simulink subsystem "Integrator_dyn_sat"  (R2022b)
settings: Solver=VariableStepAuto  StartTime=0.0  StopTime=10.0  RelTol=1e-3
model mask{initValue=0, T_s=-1}
undefined symbols (not defined in the file or in its folder): DiscIntNeverNeededParam
libraries: simulink x10
settings Model: Creator=winkens  LastModifiedBy=winkens
settings SolverCC: AlgebraicLoopSolver=TrustRegion
settings DebuggingCC: UnconnectedInputMsg=warning  UnconnectedOutputMsg=warning  UnconnectedLineMsg=warning  SFMachineParentedDataDiag=warning
settings ModelReferenceCC: EnableRefExpFcnMdlSchedulingChecks=on
settings RTWCC: DLArmComputeVersion=19.05

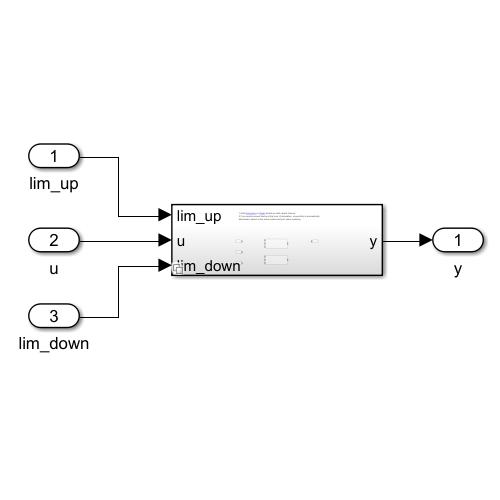
[thumbnail: Simulink's stored preview of the top-level diagram]
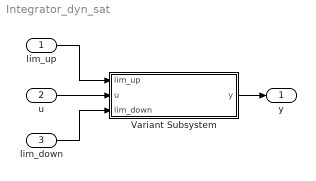
== system Integrator_dyn_sat ==
  lim_up : Inport
  u : Inport  Port=2
  lim_down : Inport  Port=3
  Variant Subsystem : Subsystem  Variant=on
  y : Outport
  wires:
  lim_up/1 -> Variant Subsystem/1(lim_up)
  lim_down/1 -> Variant Subsystem/3(lim_down)
  u/1 -> Variant Subsystem/2(u)
  Variant Subsystem/1(y) -> y/1

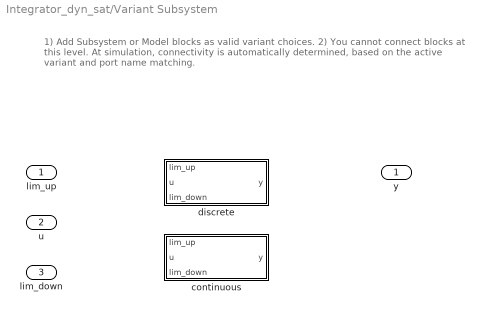
== system Integrator_dyn_sat/Variant Subsystem ==
  note: 1) Add Subsystem or Model blocks as valid variant choices.
      | 2) You cannot connect blocks at this level. At simulation, connectivity is automatically
      | determined, based on the active variant and port name matching.
  lim_up : Inport
  u : Inport  Port=2
  lim_down : Inport  Port=3
  continuous : Subsystem  VariantControl=T_s == 0
  discrete : Subsystem  VariantControl=(default)
  y : Outport

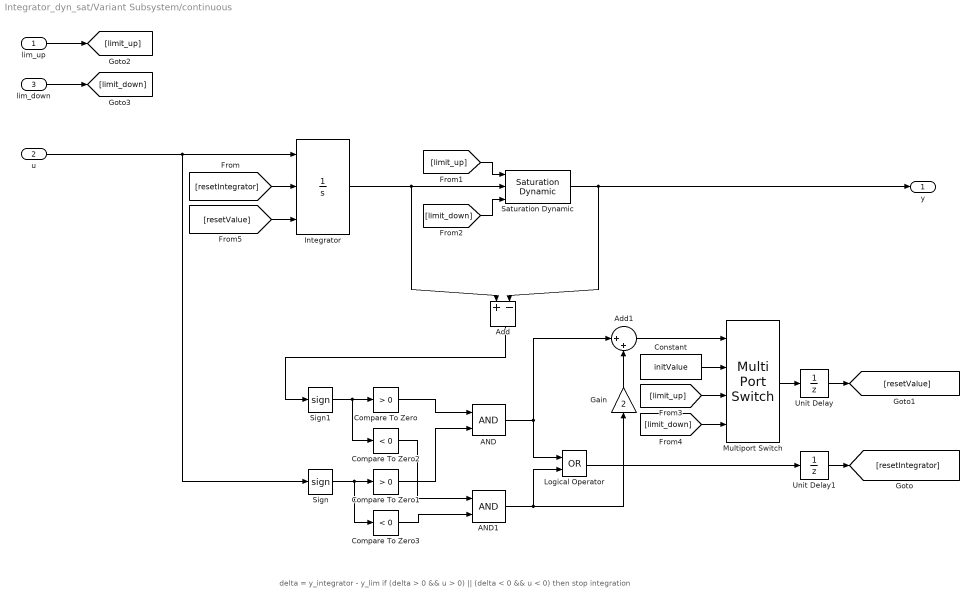
== system Integrator_dyn_sat/Variant Subsystem/continuous ==
  note: delta = y_integrator - y_lim
      |
      | if (delta > 0 && u > 0) || (delta < 0 && u < 0) then stop integration
  lim_up : Inport
  u : Inport  Port=2
  lim_down : Inport  Port=3
  AND : Logic  AllPortsSameDT=off  OutDataTypeStr=boolean
  AND1 : Logic  AllPortsSameDT=off  OutDataTypeStr=boolean
  Add : Sum  Inputs=+-
  Add1 : Sum  Inputs=|++
  Compare To Zero : simulink/Logic and Bit Operations/Compare To Zero  relop=>  OutDataTypeStr=boolean
  Compare To Zero1 : simulink/Logic and Bit Operations/Compare To Zero  relop=>  OutDataTypeStr=boolean
  Compare To Zero2 : simulink/Logic and Bit Operations/Compare To Zero  relop=<  OutDataTypeStr=boolean
  Compare To Zero3 : simulink/Logic and Bit Operations/Compare To Zero  relop=<  OutDataTypeStr=boolean
  Constant : Constant  Value=initValue
  Gain : Gain  Gain=2
  Integrator : Integrator  ExternalReset=level hold  InitialConditionSource=external
  Logical Operator : Logic  Operator=OR  AllPortsSameDT=off  OutDataTypeStr=boolean
  Multiport Switch : MultiPortSwitch  DataPortOrder=Zero-based contiguous  zeroidx=on  SaturateOnIntegerOverflow=off  InputSameDT=off
  Saturation Dynamic : simulink/Discontinuities/Saturation Dynamic  OutMin=[]  OutMax=[]  OutDataTypeStr=Inherit: Same as second input  OutDataType=fixdt(1, 16)  OutScaling=2^-10  DoSatur=off
  Sign : Signum
  Sign1 : Signum
  Unit Delay : UnitDelay  InitialCondition=initValue  SampleTime=-1  HasFrameUpgradeWarning=on
  Unit Delay1 : UnitDelay  SampleTime=-1  HasFrameUpgradeWarning=on
  y : Outport
  wires:
  Unit Delay1/1 -> [resetIntegrator]
  Unit Delay/1 -> [resetValue]
  u/1 -> Integrator/1, Sign/1
  Add/1 -> Sign1/1
  Compare To Zero2/1 -> AND1/1
  Gain/1 -> Add1/2
  Saturation Dynamic/1 -> y/1, Add/2
  Integrator/1 -> Add/1, Saturation Dynamic/2
  [resetValue] -> Integrator/3
  Compare To Zero1/1 -> AND/2
  Logical Operator/1 -> Unit Delay1/1
  Compare To Zero/1 -> AND/1
  [limit_down] -> Saturation Dynamic/3
  AND1/1 -> Logical Operator/2, Gain/1
  lim_down/1 -> [limit_down]
  [limit_up] -> Saturation Dynamic/1
  Sign1/1 -> Compare To Zero/1, Compare To Zero2/1
  Compare To Zero3/1 -> AND1/2
  AND/1 -> Logical Operator/1, Add1/1
  Sign/1 -> Compare To Zero1/1, Compare To Zero3/1
  Constant/1 -> Multiport Switch/2
  Multiport Switch/1 -> Unit Delay/1
  Add1/1 -> Multiport Switch/1
  [resetIntegrator] -> Integrator/2
  [limit_down] -> Multiport Switch/4
  [limit_up] -> Multiport Switch/3
  lim_up/1 -> [limit_up]

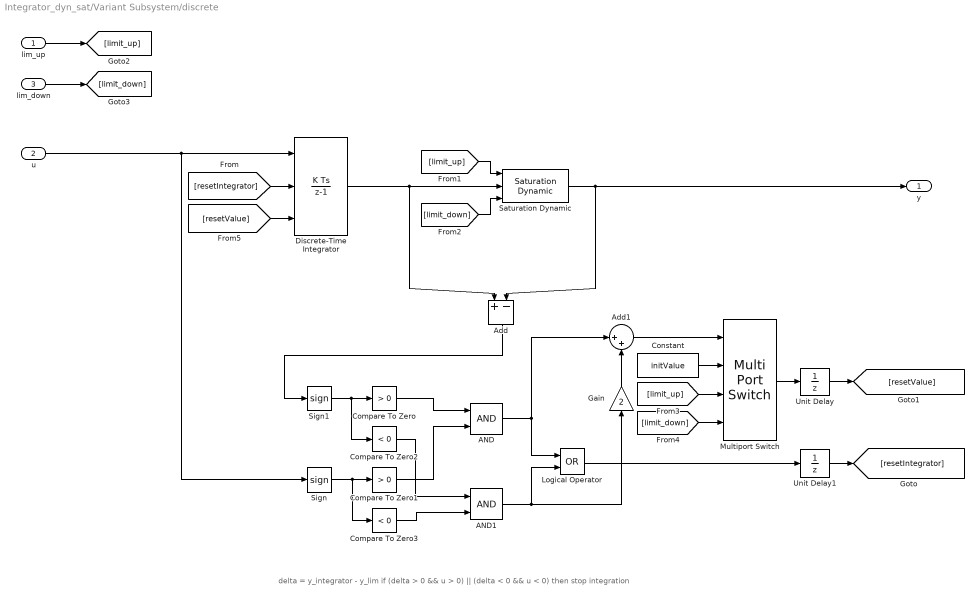
== system Integrator_dyn_sat/Variant Subsystem/discrete ==
  note: delta = y_integrator - y_lim
      |
      | if (delta > 0 && u > 0) || (delta < 0 && u < 0) then stop integration
  lim_up : Inport
  u : Inport  Port=2
  lim_down : Inport  Port=3
  AND : Logic  AllPortsSameDT=off  OutDataTypeStr=boolean
  AND1 : Logic  AllPortsSameDT=off  OutDataTypeStr=boolean
  Add : Sum  Inputs=+-
  Add1 : Sum  Inputs=|++
  Compare To Zero : simulink/Logic and Bit Operations/Compare To Zero  relop=>  OutDataTypeStr=boolean
  Compare To Zero1 : simulink/Logic and Bit Operations/Compare To Zero  relop=>  OutDataTypeStr=boolean
  Compare To Zero2 : simulink/Logic and Bit Operations/Compare To Zero  relop=<  OutDataTypeStr=boolean
  Compare To Zero3 : simulink/Logic and Bit Operations/Compare To Zero  relop=<  OutDataTypeStr=boolean
  Constant : Constant  Value=initValue
  Discrete-Time Integrator : DiscreteIntegrator  ExternalReset=sampled level  InitialConditionSource=external  InitialCondition=initValue  SampleTime=T_s  ICPrevOutput=DiscIntNeverNeededParam  ICPrevScaledInput=DiscIntNeverNeededParam
  Gain : Gain  Gain=2
  Logical Operator : Logic  Operator=OR  AllPortsSameDT=off  OutDataTypeStr=boolean
  Multiport Switch : MultiPortSwitch  DataPortOrder=Zero-based contiguous  zeroidx=on  SaturateOnIntegerOverflow=off  InputSameDT=off
  Saturation Dynamic : simulink/Discontinuities/Saturation Dynamic  OutMin=[]  OutMax=[]  OutDataTypeStr=Inherit: Same as second input  OutDataType=fixdt(1, 16)  OutScaling=2^-10  DoSatur=off
  Sign : Signum
  Sign1 : Signum
  Unit Delay : UnitDelay  InitialCondition=initValue  SampleTime=-1  HasFrameUpgradeWarning=on
  Unit Delay1 : UnitDelay  SampleTime=-1  HasFrameUpgradeWarning=on
  y : Outport
  wires:
  Unit Delay1/1 -> [resetIntegrator]
  Unit Delay/1 -> [resetValue]
  u/1 -> Discrete-Time Integrator/1, Sign/1
  Add/1 -> Sign1/1
  [resetValue] -> Discrete-Time Integrator/3
  [limit_down] -> Multiport Switch/4
  [limit_up] -> Multiport Switch/3
  [limit_down] -> Saturation Dynamic/3
  [limit_up] -> Saturation Dynamic/1
  lim_down/1 -> [limit_down]
  lim_up/1 -> [limit_up]
  Constant/1 -> Multiport Switch/2
  Gain/1 -> Add1/2
  Add1/1 -> Multiport Switch/1
  Multiport Switch/1 -> Unit Delay/1
  [resetIntegrator] -> Discrete-Time Integrator/2
  Logical Operator/1 -> Unit Delay1/1
  Sign/1 -> Compare To Zero1/1, Compare To Zero3/1
  Sign1/1 -> Compare To Zero/1, Compare To Zero2/1
  AND1/1 -> Logical Operator/2, Gain/1
  AND/1 -> Logical Operator/1, Add1/1
  Compare To Zero3/1 -> AND1/2
  Compare To Zero2/1 -> AND1/1
  Compare To Zero1/1 -> AND/2
  Compare To Zero/1 -> AND/1
  Discrete-Time Integrator/1 -> Add/1, Saturation Dynamic/2
  Saturation Dynamic/1 -> y/1, Add/2
